simulink model "tractor_mu2018"  (R2018a)
settings: Solver=FixedStepDiscrete  StartTime=0.0  StopTime=30  FixedStep=0.001  RelTol=1e-3
model workspace (MAT data in the model file):
  MCOS : class17 (value not decoded)
undefined symbols (not defined in the file): A, a, B, b, C, D, DiscIntNeverNeededParam, Iz, K, k1, K1, k2, K2, L1, L2, m, magnitude, Phi, Sample_time, Steer_Ratio
libraries: simulink x39, Solver_SF x1, dsparch4 x1
(part 2 of 5)

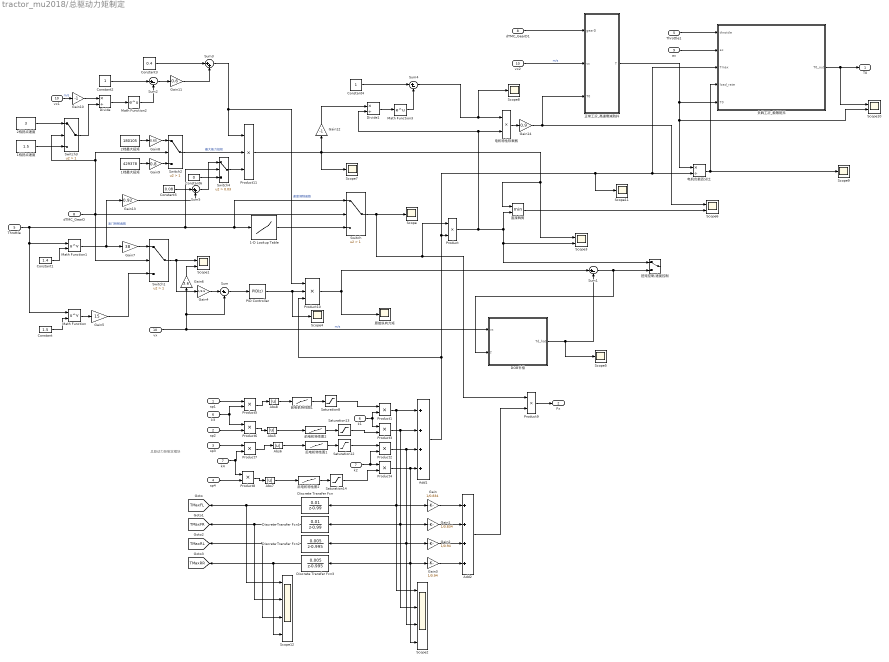
== system tractor_mu2018/总驱动力矩制定 ==
  note: 总驱动力矩制定模块
  sp1 : Inport
  sp2 : Inport  Port=2
  sp3 : Inport  Port=3
  sp4 : Inport  Port=4
  Throttle : Inport  Port=5
  k1 : Inport  Port=6
  k2 : Inport  Port=7
  dTMC_GearD : Inport  Port=8
  ax : Inport  Port=9
  vx : Inport  Port=10
  1-D Lookup Table : Lookup_n-D  NumberOfTableDimensions=1  BreakpointsForDimension1=[0 0.1 0.2 0.3 0.4 0.5 0.6 0.7 0.8 0.9 1]  Table=[0 0.02 0.04 0.09 0.14 0.23 0.32 0.46 0.6 0.8 1]  InternalRulePriority=Speed  RndMeth=Simplest  InputSameDT=on
  1档拐点速度 : Constant  Value=1.5
  1档最大扭矩 : Constant  Value=429378
  2档拐点速度 : Constant  Value=3
  2档最大扭矩 : Constant  Value=180105
  Abs{5..8} (4 alike) : Abs
  Add1 : Sum  Inputs=++++
  Add2 : Sum  Inputs=++++
  Constant : Constant  Value=1.5
  Constant1 : Constant  Value=1.4
  Constant2 : Constant
  Constant3 : Constant  Value=0.4
  Constant4 : Constant
  Constant5 : Constant  Value=0.08
  Constant6 : Constant  Value=0
  DOB补偿 : Subsystem
  Discrete Transfer Fcn : DiscreteTransferFcn  Numerator=[0.01]  Denominator=[1 -0.99]
  Discrete Transfer Fcn1 : DiscreteTransferFcn  Numerator=[0.01]  Denominator=[1 -0.99]
  Discrete Transfer Fcn2 : DiscreteTransferFcn  Numerator=[0.005]  Denominator=[1 -0.995]
  Discrete Transfer Fcn3 : DiscreteTransferFcn  Numerator=[0.005]  Denominator=[1 -0.995]
  Divide : Product  Inputs=*/
  Divide1 : Product  Inputs=*/
  Gain : Gain  Gain=1/0.834
  Gain1 : Gain  Gain=1/0.834
  Gain10 : Gain  Gain=-1
  Gain11 : Gain  Gain=0.6
  Gain12 : Gain  Gain=-1
  Gain13 : Gain  Gain=0.92
  Gain14 : Gain  Gain=0.9
  Gain2 : Gain  Gain=1/0.94
  Gain3 : Gain  Gain=1/0.94
  Gain4 : Gain  Gain=1/3.6
  Gain5 : Gain  Gain=15
  Gain6 : Gain  Gain=3.6
  Gain7 : Gain  Gain=38
  Gain8 : Gain  Gain=0.65
  Gain9 : Gain  Gain=0.8
  Math Function : Math  Operator=pow  SaturateOnIntegerOverflow=on
  Math Function1 : Math  Operator=pow  SaturateOnIntegerOverflow=on
  Math Function2 : Math  SaturateOnIntegerOverflow=on
  Math Function3 : Math  SaturateOnIntegerOverflow=on
  PID Controller : simulink/Continuous/PID Controller  Controller=PID  Form=Parallel  TimeDomain=Discrete-time  SampleTime=-1  IntegratorMethod=Forward Euler  FilterMethod=Forward Euler  ControllerParametersSource=internal  P=0.3  I=0.1  D=0  N=100  UseFilter=on  TunerSelectOption=Transfer Function Based (PID Tuner App)  InitialConditionSource=internal  InitialConditionForIntegrator=0  InitialConditionForFilter=0  DifferentiatorICPrevScaledInput=0  ExternalReset=none  TrackingMode=off  Kt=1  LimitOutput=on  UpperSaturationLimit=1  LowerSaturationLimit=0  LinearizeAsGain=on  AntiWindupMode=none  Kb=1  POutMin=[]  POutMax=[]  IOutMin=[]  IOutMax=[]  DOutMin=[]  DOutMax=[]  NOutMin=[]  NOutMax=[]  SumOutMin=[]  SumOutMax=[]  SaturationOutMin=[]  SaturationOutMax=[]  PParamMin=[]  PParamMax=[]  IParamMin=[]  IParamMax=[]  DParamMin=[]  DParamMax=[]  NParamMin=[]  NParamMax=[]  KbParamMin=[]  KbParamMax=[]  KtParamMin=[]  KtParamMax=[]  KbOutMin=[]  KbOutMax=[]  KtOutMin=[]  KtOutMax=[]  IntegratorOutMin=[]  IntegratorOutMax=[]  FilterOutMin=[]  FilterOutMax=[]  SumI1OutMin=[]  SumI1OutMax=[]  SumI2OutMin=[]  SumI2OutMax=[]  SumI3OutMin=[]  SumI3OutMax=[]  SumDOutMin=[]  SumDOutMax=[]  DifferentiatorOutMin=[]  DifferentiatorOutMax=[]  FilterDiffOutCoefMin=[]  FilterDiffOutCoefMax=[]  ReciprocalOutMin=[]  ReciprocalOutMax=[]  SumDenOutMin=[]  SumDenOutMax=[]  SumNumOutMin=[]  SumNumOutMax=[]  DivideOutMin=[]  DivideOutMax=[]  IntegratorContinuousStateAttributes=''  IntegratorStateMustResolveToSignalObject=off  IntegratorRTWStateStorageClass=Auto  FilterContinuousStateAttributes=''  FilterStateMustResolveToSignalObject=off  FilterRTWStateStorageClass=Auto
  Product{,1..9} (10 alike) : Product
  Product10 : Product  Inputs=3
  Product11 : Product  Inputs=3
  Saturation12 : Saturate  UpperLimit=1800  LowerLimit=0
  Saturation13 : Saturate  UpperLimit=1100  LowerLimit=0
  Saturation14 : Saturate  UpperLimit=1800  LowerLimit=0
  Saturation8 : Saturate  UpperLimit=1100  LowerLimit=0
  Scope{,4..5,7..9,11} (7 alike) : Scope
  Scope{1,3,6,10} (4 alike) : Scope  NumInputPorts=2
  Scope12 : Scope  NumInputPorts=4
  Scope2 : Scope  NumInputPorts=4
  Sum{,1..2,4} (4 alike) : Sum  Inputs=|+-
  Sum3 : Sum  Inputs=|++
  Sum5 : Sum  Inputs=|++
  Switch{,1..3} (4 alike) : Switch  Criteria=u2 > Threshold  Threshold=1
  Switch4 : Switch  Criteria=u2 > Threshold  Threshold=0.03
  Throttle1 : InportShadow  Port=5
  dTMC_GearD1 : InportShadow  Port=8
  k3 : InportShadow  Port=6
  k4 : InportShadow  Port=7
  vx1 : InportShadow  Port=10
  vx2 : InportShadow  Port=10
  前电机特性图1 : Lookup_n-D  NumberOfTableDimensions=1  BreakpointsForDimension1=[0;600;900;1200;1500;1800;2104;2402;2701;3001;3302;3600;3901;4200;4501;4801;5000;5001]  Table=[1116;1107;1102;1099;1101;913;734;611;523;456;403;363;327;305;278;253;240;0]  InternalRulePriority=Speed  OutMin=0  OutMax=1200  RndMeth=Simplest  InputSameDT=on
  前电机特性图2 : Lookup_n-D  NumberOfTableDimensions=1  BreakpointsForDimension1=[0;600;900;1200;1500;1800;2104;2402;2701;3001;3302;3600;3901;4200;4501;4801;5000;5001]  Table=[1116;1107;1102;1099;1101;913;734;611;523;456;403;363;327;305;278;253;240;0]  InternalRulePriority=Speed  OutMin=0  OutMax=1200  RndMeth=Simplest  InputSameDT=on
  原始纵向力矩 : Scope
  后电机特性图1 : Lookup_n-D  NumberOfTableDimensions=1  BreakpointsForDimension1=[0;299;599.6;899.7;1200;1500;1800;2099;2399.4;2698.5;2998.1;3300;3599;3899;4197.8;4201]  Table=[1868;1868.3;1868.6;1844.3;1842.3;1763.9;1516.4;1277.9;1098.6;954;839.4;727;645.7;585.53;529.7;0]  InternalRulePriority=Speed  OutMin=[0]  OutMax=[1800]  RndMeth=Simplest  InputSameDT=on
  后电机特性图2 : Lookup_n-D  NumberOfTableDimensions=1  BreakpointsForDimension1=[0;500;1000;1200;1600;2000;2800;3200;3600;4200;4201]  Table=[1800;1800;1800;1800;1700;1360;900;750;650;520;0]  InternalRulePriority=Speed  OutMin=[0]  OutMax=[1800]  RndMeth=Simplest  InputSameDT=on
  扭矩控制/速度控制 : ManualSwitch
  正常工况_高速衰减防抖 : Subsystem
  电机特性软裁剪 : Product
  电机负载百分比 : Product  Inputs=*/
  直接裁剪 : MinMax  Inputs=2
  负载工况_极限防抖 : Stateflow chart  TreatAsAtomicUnit=on
  T0 : Outport
  Fx : Outport  Port=2
  tag scope: TMaxFL=global, TMaxFR=global, TMaxRL=global, TMaxRR=global
  wires:
  sp3/1 -> Product7/1
  Saturation8/1 -> Product1/1
  前电机特性图2/1 -> Saturation13/1
  后电机特性图1/1 -> Saturation12/1
  sp1/1 -> Product5/1
  sp4/1 -> Product8/2
  Abs7/1 -> 后电机特性图2/1
  Product2/1 -> Discrete Transfer Fcn2/1, Scope2/3, Gain2/1, Add1/3
  前电机特性图1/1 -> Saturation8/1
  sp2/1 -> Product6/2
  Product3/1 -> Add1/2, Discrete Transfer Fcn1/1, Scope2/2, Gain1/1
  后电机特性图2/1 -> Saturation14/1
  Saturation12/1 -> Product2/1
  Abs5/1 -> 前电机特性图2/1
  Abs6/1 -> 后电机特性图1/1
  Abs8/1 -> 前电机特性图1/1
  k1/1 -> Product3/1, Product1/2
  Saturation13/1 -> Product3/2
  k2/1 -> Product4/1, Product2/2
  Saturation14/1 -> Product4/2
  Product4/1 -> Discrete Transfer Fcn3/1, Scope2/4, Gain3/1, Add1/4
  Product/1 -> Divide1/2, 电机特性软裁剪/2, 直接裁剪/2, Scope3/2, 扭矩控制/速度控制/1
  k3/1 -> Product6/1, Product5/2
  Product5/1 -> Abs8/1
  Product6/1 -> Abs5/1
  k4/1 -> Product8/1, Product7/2
  Product7/1 -> Abs6/1
  Product8/1 -> Abs7/1
  1-D Lookup Table/1 -> Switch/3
  Gain/1 -> Add2/1
  Gain1/1 -> Add2/2
  Gain2/1 -> Add2/3
  Gain3/1 -> Add2/4
  Add2/1 -> Product9/2
  Product9/1 -> Fx/1
  Throttle/1 -> Math Function/1, Math Function1/1, Switch4/2, Switch/1, 1-D Lookup Table/1
  Constant/1 -> Math Function/2
  Math Function/1 -> Gain5/1
  Gain5/1 -> Switch1/3
  Constant1/1 -> Math Function1/2
  Gain7/1 -> Switch1/1
  Math Function1/1 -> Gain13/1, Gain7/1  "油门映射函数"
  Switch1/1 -> Gain4/1, Scope1/1
  Gain4/1 -> Sum/1
  vx/1 -> Sum/2, Gain6/1, DOB补偿/1(vx)  "m/s"
  Switch/1 -> Product9/1, Product/1, Scope/1
  Sum/1 -> PID Controller/1
  PID Controller/1 -> Scope4/1, Product10/2
  Product10/1 -> Sum1/1, 原始纵向力矩/1
  Gain6/1 -> Scope1/2
  Sum1/1 -> DOB补偿/2(T), 扭矩控制/速度控制/2
  DOB补偿/1(Td_hat) -> Scope5/1, Sum1/2
  1档最大扭矩/1 -> Gain9/1
  2档最大扭矩/1 -> Gain8/1
  Gain8/1 -> Switch2/1
  Gain9/1 -> Switch2/3
  Switch2/1 -> Product11/2  "最大能力扭矩"
  Constant2/1 -> Sum2/1
  Math Function2/1 -> Sum2/2
  1档拐点速度/1 -> Switch3/3
  2档拐点速度/1 -> Switch3/1
  dTMC_GearD/1 -> Switch3/2, Switch2/2, Switch1/2, Switch/2
  vx1/1 -> Gain10/1  "m/s"
  Switch3/1 -> Divide/2
  Gain10/1 -> Divide/1
  Divide/1 -> Math Function2/1
  Sum2/1 -> Gain11/1
  Constant3/1 -> Sum3/1
  Gain11/1 -> Sum3/2
  Sum3/1 -> Product10/1, Product11/1  "速度调制函数"
  Constant4/1 -> Sum4/1
  Math Function3/1 -> Sum4/2
  Divide1/1 -> Math Function3/1
  Gain12/1 -> Divide1/1
  Sum4/1 -> Scope8/1, 电机特性软裁剪/1
  Product11/1 -> Scope7/1, 直接裁剪/1, Scope3/1, Gain12/1
  Sum5/1 -> Switch4/1
  Gain13/1 -> Sum5/2
  Constant5/1 -> Sum5/1
  Switch4/1 -> Product11/3
  Constant6/1 -> Switch4/3
  电机特性软裁剪/1 -> Gain14/1
  直接裁剪/1 -> Scope6/2
  Product1/1 -> Discrete Transfer Fcn/1, Scope2/1, Gain/1, Add1/1
  dTMC_GearD1/1 -> 正常工况_高速衰减防抖/1(gearD)
  vx2/1 -> 正常工况_高速衰减防抖/2(vx)  "m/s"
  Throttle1/1 -> 负载工况_极限防抖/1(throttle)
  ax/1 -> 负载工况_极限防抖/2(ax)
  Add1/1 -> Scope11/1, 负载工况_极限防抖/3(Tmax), 电机负载百分比/2, Product/2, Product10/3
  正常工况_高速衰减防抖/1(T) -> 负载工况_极限防抖/5(T0), Scope10/2, 电机负载百分比/1
  电机负载百分比/1 -> 负载工况_极限防抖/4(load_rate), Scope9/1
  负载工况_极限防抖/1(T0_out) -> Scope10/1, T0/1
  Discrete Transfer Fcn/1 -> Scope12/1, [TMaxFL]
  Discrete Transfer Fcn1/1 -> Scope12/2, [TMaxFR]
  Discrete Transfer Fcn2/1 -> Scope12/3, [TMaxRL]
  Discrete Transfer Fcn3/1 -> Scope12/4, [TMaxRR]
  Gain14/1 -> Scope6/1, 正常工况_高速衰减防抖/3(T0)

== system tractor_mu2018/挡位与刹车处理1 ==
  dTMC_GearD : Inport
  Constant6 : Constant  Value=15.88
  Constant7 : Constant  Value=30.6204
  Constant8 : Constant  Value=63.52
  Constant9 : Constant  Value=80.454
  Switch2 : Switch  Criteria=u2 > Threshold  Threshold=1
  Switch3 : Switch  Criteria=u2 > Threshold  Threshold=1
  spdratio_F : Outport
  spdratio_R : Outport  Port=2
  wires:
  Switch3/1 -> spdratio_R/1
  Constant9/1 -> Switch3/3
  Switch2/1 -> spdratio_F/1
  Constant8/1 -> Switch2/3
  dTMC_GearD/1 -> Switch3/2, Switch2/2
  Constant6/1 -> Switch2/1
  Constant7/1 -> Switch3/1

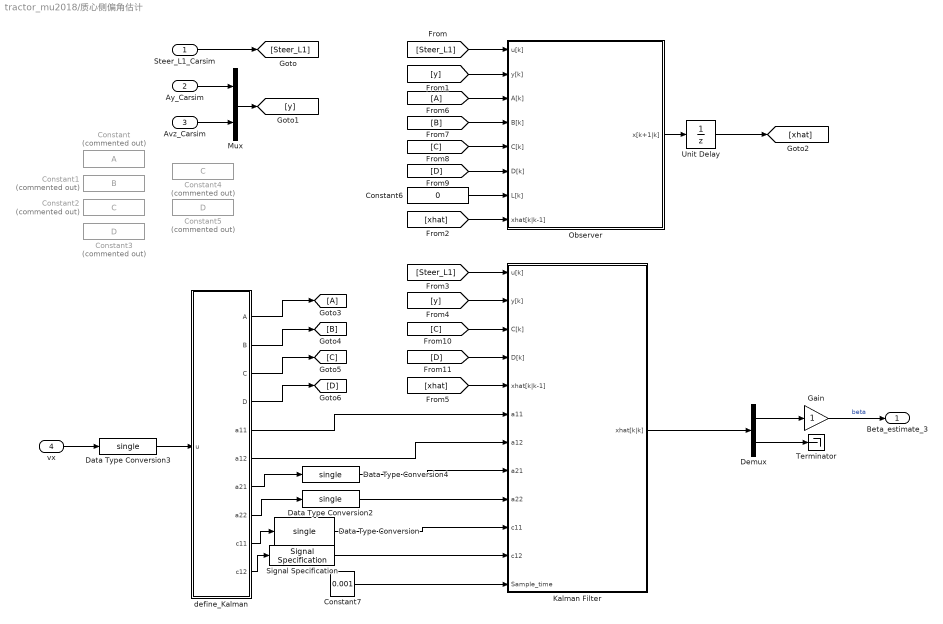
== system tractor_mu2018/质心侧偏角估计 ==
  Steer_L1_Carsim : Inport
  Ay_Carsim : Inport  Port=2
  Avz_Carsim : Inport  Port=3
  vx : Inport  Port=4
  Constant : Constant  Commented=on  Value=A
  Constant1 : Constant  Commented=on  Value=B
  Constant2 : Constant  Commented=on  Value=C
  Constant3 : Constant  Commented=on  Value=D
  Constant4 : Constant  Commented=on  Value=C
  Constant5 : Constant  Commented=on  Value=D
  Constant6 : Constant  Value=0
  Constant7 : Constant  Value=0.001  OutDataTypeStr=single
  Data Type Conversion{,2..4} (4 alike) : DataTypeConversion  OutDataTypeStr=single
  Demux : Demux  Outputs=2
  Gain : Gain
  Kalman Filter : Subsystem
  Mux : Mux  Inputs=2
  Observer : Subsystem
  Signal Specification : SignalSpecification  OutDataTypeStr=single
  Terminator : Terminator
  Unit Delay : UnitDelay  SampleTime=-1  HasFrameUpgradeWarning=on
  define_Kalman : MATLAB Function  TreatAsAtomicUnit=on
  Beta_estimate_3 : Outport
  wires:
  Steer_L1_Carsim/1 -> [Steer_L1]
  Ay_Carsim/1 -> Mux/1
  Avz_Carsim/1 -> Mux/2
  Mux/1 -> [y]
  [Steer_L1] -> Observer/1(u[k])
  [y] -> Observer/2(y[k])
  Observer/1(x[k+1|k]) -> Unit Delay/1
  Unit Delay/1 -> [xhat]
  [xhat] -> Observer/8(xhat[k|k-1])
  [Steer_L1] -> Kalman Filter/1(u[k])
  [y] -> Kalman Filter/2(y[k])
  [xhat] -> Kalman Filter/5(xhat[k|k-1])
  Demux/1 -> Gain/1
  Demux/2 -> Terminator/1
  Constant6/1 -> Observer/7(L[k])
  vx/1 -> Data Type Conversion3/1
  define_Kalman/1(A) -> [A]
  define_Kalman/2(B) -> [B]
  define_Kalman/3(C) -> [C]
  define_Kalman/4(D) -> [D]
  [A] -> Observer/3(A[k])
  [B] -> Observer/4(B[k])
  [C] -> Observer/5(C[k])
  [D] -> Observer/6(D[k])
  [C] -> Kalman Filter/3(C[k])
  [D] -> Kalman Filter/4(D[k])
  Constant7/1 -> Kalman Filter/12(Sample_time)
  define_Kalman/10(c12) -> Signal Specification/1
  define_Kalman/9(c11) -> Data Type Conversion/1
  define_Kalman/8(a22) -> Data Type Conversion2/1
  define_Kalman/6(a12) -> Kalman Filter/7(a12)
  define_Kalman/5(a11) -> Kalman Filter/6(a11)
  Signal Specification/1 -> Kalman Filter/11(c12)
  Data Type Conversion3/1 -> define_Kalman/1(u)
  define_Kalman/7(a21) -> Data Type Conversion4/1
  Data Type Conversion2/1 -> Kalman Filter/9(a22)
  Data Type Conversion/1 -> Kalman Filter/10(c11)
  Kalman Filter/1(xhat[k|k]) -> Demux/1
  Data Type Conversion4/1 -> Kalman Filter/8(a21)
  Gain/1 -> Beta_estimate_3/1  "beta"

== system tractor_mu2018/质心侧偏角滑模观测器估计 ==
  Steer_L1_Carsim : Inport
  Avz_Carsim : Inport  Port=2
  vx : Inport  Port=3
  Subsystem : Subsystem
  Subsystem1 : Subsystem  Commented=on
  delta_f : Gain  Gain=1/Steer_Ratio
  beta_est : Outport
  gamma_est : Outport  Port=2
  vy_hat_out : Outport  Port=3
  wires:
  Steer_L1_Carsim/1 -> delta_f/1
  Avz_Carsim/1 -> Subsystem/1(Avz_Carsim)
  vx/1 -> Subsystem/2(vx)
  delta_f/1 -> Subsystem/3(delta_f)
  Subsystem/1(beta_est) -> beta_est/1
  Subsystem/2(gamma_est) -> gamma_est/1
  Subsystem/3(vy_hat_output) -> vy_hat_out/1

== system tractor_mu2018/质心侧偏角观测 ==
  前轮转角 : Inport
  前轮纵向力 : Inport  Port=2
  后轮纵向力 : Inport  Port=3
  纵向速度 : Inport  Port=4
  横摆角速度 : Inport  Port=5
  Demux : Demux  Outputs=3
  Gain : Gain  Gain=0.001
  MATLAB Function : MATLAB Function  TreatAsAtomicUnit=on
  Mux : Mux  Inputs=3
  Mux1 : Mux  Inputs=2
  Scope : Scope
  Scope1 : Scope
  Sum : Sum  Inputs=|++
  Sum1 : Sum  Inputs=|+-
  Unit Delay : UnitDelay  InitialCondition=[0.1;0;0]  SampleTime=0.001  HasFrameUpgradeWarning=on
  Unit Delay1 : UnitDelay  InitialCondition=[0.1;0;0]  SampleTime=0.001  HasFrameUpgradeWarning=on
  估计横摆角速度 : Scope
  估计纵向速度 : Scope
  侧偏角估计 : Scope
  侧偏角 : Outport
  纵向速度估计 : Outport  Port=2
  横摆角速度估计 : Outport  Port=3
  wires:
  MATLAB Function/1(x_dot) -> Scope1/1, Gain/1
  Gain/1 -> Sum/1
  Unit Delay/1 -> Sum/2
  Sum/1 -> Unit Delay1/1, Demux/1, Unit Delay/1
  Demux/2 -> 侧偏角估计/1, 侧偏角/1
  Demux/1 -> 纵向速度估计/1, 估计纵向速度/1
  Demux/3 -> 横摆角速度估计/1, 估计横摆角速度/1
  前轮转角/1 -> Mux/1
  前轮纵向力/1 -> Mux/2
  后轮纵向力/1 -> Mux/3
  Mux/1 -> MATLAB Function/2(u)
  纵向速度/1 -> Mux1/1
  横摆角速度/1 -> Mux1/2
  Mux1/1 -> Sum1/1, MATLAB Function/3(z_meas)
  MATLAB Function/2(z_hat) -> Sum1/2
  Sum1/1 -> Scope/1
  Unit Delay1/1 -> MATLAB Function/1(x_hat)

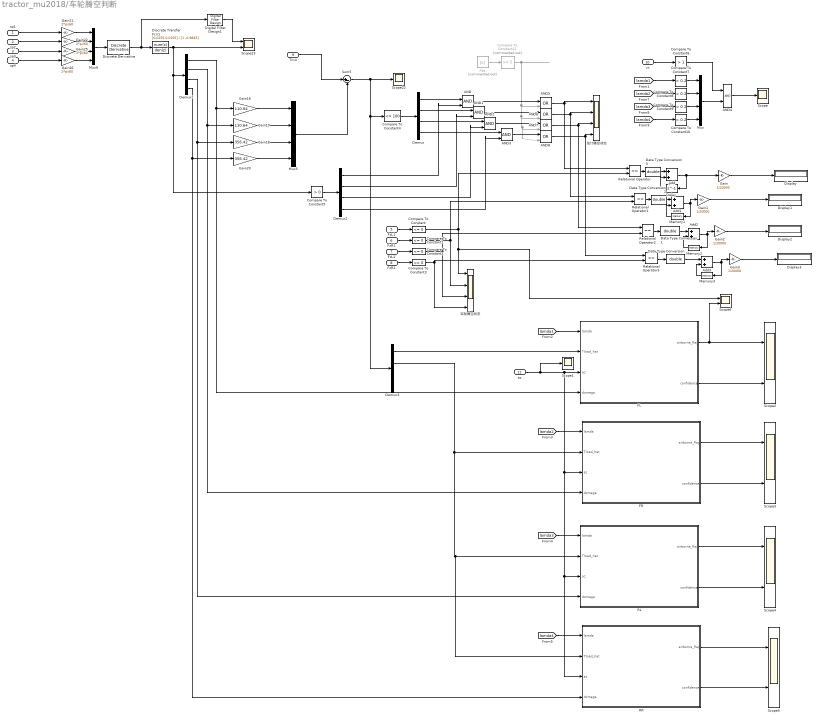
== system tractor_mu2018/车轮腾空判断 ==
  sp1 : Inport
  sp2 : Inport  Port=2
  sp3 : Inport  Port=3
  sp4 : Inport  Port=4
  FzL1 : Inport  Port=5
  FzR1 : Inport  Port=6
  FzL2 : Inport  Port=7
  FzR2 : Inport  Port=8
  Tm4 : Inport  Port=9
  vx : Inport  Port=10
  az : Inport  Port=11
  AND{,1..4} (5 alike) : Logic  IconShape=distinctive  AllPortsSameDT=off  OutDataTypeStr=boolean
  AND{5..8} (4 alike) : Logic  Operator=OR  IconShape=distinctive  AllPortsSameDT=off  OutDataTypeStr=boolean
  Abs : Abs  Commented=on
  Add : Sum
  Add1 : Sum
  Add2 : Sum
  Add3 : Sum  AccumDataTypeStr=double
  Compare To Constant{,1..3} (4 alike) : simulink/Logic and Bit Operations/Compare To Constant  relop=<=  const=0  OutDataTypeStr=boolean
  Compare To Constant{7..10} (4 alike) : simulink/Logic and Bit Operations/Compare To Constant  relop=>  const=0.2  OutDataTypeStr=boolean
  Compare To Constant11 : simulink/Logic and Bit Operations/Compare To Constant  Commented=on  relop=>=  const=5  OutDataTypeStr=boolean
  Compare To Constant4 : simulink/Logic and Bit Operations/Compare To Constant  relop=<=  const=100  OutDataTypeStr=boolean
  Compare To Constant5 : simulink/Logic and Bit Operations/Compare To Constant  relop=>  const=0  OutDataTypeStr=boolean
  Compare To Constant6 : simulink/Logic and Bit Operations/Compare To Constant  relop=>  const=1  OutDataTypeStr=boolean
  Data Type Conversion{,1..3} (4 alike) : DataTypeConversion  OutDataTypeStr=double
  Delay : Delay  DelayLength=1
  Demux{,1..3} (4 alike) : Demux
  Digital Filter Design1 : dsparch4/Digital Filter Design  mwdsp_browser_bugfix_var=off
  Discrete Transfer Fcn1 : DiscreteTransferFcn  Numerator=[0.0155 0.0155]  Denominator=[1 -0.9845]
  Discrete Derivative : simulink/Discrete/Discrete Derivative  gainval=1.0  ICPrevScaledInput=0.0  OutMin=[]  OutMax=[]  OutDataType=fixdt(1, 16)  OutScaling=2^-10  DoSatur=off
  Display{,1..3} (4 alike) : Display
  FL : Stateflow chart  TreatAsAtomicUnit=on
  FR : Stateflow chart  TreatAsAtomicUnit=on
  Gain{,1..3} (4 alike) : Gain  Gain=1/20000
  Gain16 : Gain  Gain=110.64
  Gain18 : Gain  Gain=356.42
  Gain19 : Gain  Gain=110.64
  Gain20 : Gain  Gain=356.42
  Gain{21..22,25..26} (4 alike) : Gain  Gain=2*pi/60
  Memory1 : Memory
  Memory2 : Memory
  Memory3 : Memory
  Mux : Mux
  Mux5 : Mux
  Mux6 : Mux
  RL : Stateflow chart  TreatAsAtomicUnit=on
  RR : Stateflow chart  TreatAsAtomicUnit=on
  Relational Operator{,1..3} (4 alike) : RelationalOperator  Operator===  OutDataTypeStr=boolean  RndMeth=Simplest
  Scope : Scope
  Scope1 : Scope
  Scope{2..6,23} (6 alike) : Scope  NumInputPorts=2
  Scope22 : Scope
  Sum5 : Sum  Inputs=|+-
  估计腾空状态 : Scope  NumInputPorts=4
  实际腾空状态 : Scope  NumInputPorts=4
  wires:
  Digital Filter Design1/1 -> Scope23/1
  Compare To Constant2/1 -> Relational Operator2/2, 实际腾空状态/3
  sp2/1 -> Gain22/1
  Discrete Transfer Fcn1/1 -> Compare To Constant5/1, Demux1/1, Scope23/2
  Compare To Constant3/1 -> Relational Operator3/2, 实际腾空状态/4
  Compare To Constant/1 -> Relational Operator/2, Scope6/1, 实际腾空状态/1
  FzL1/1 -> Compare To Constant/1
  Gain21/1 -> Mux6/1
  Mux5/1 -> Sum5/2
  Tm4/1 -> Sum5/1
  Mux6/1 -> Discrete Derivative/1
  Gain19/1 -> Mux5/2
  Gain26/1 -> Mux6/4
  Discrete Derivative/1 -> Digital Filter Design1/1, Discrete Transfer Fcn1/1
  Gain22/1 -> Mux6/2
  Compare To Constant1/1 -> Relational Operator1/2, 实际腾空状态/2
  Gain18/1 -> Mux5/3
  Gain25/1 -> Mux6/3
  Gain20/1 -> Mux5/4
  FzR2/1 -> Compare To Constant3/1
  Demux1/1 -> FL/4(domega), Gain16/1
  FzL2/1 -> Compare To Constant2/1
  Gain16/1 -> Mux5/1
  FzR1/1 -> Compare To Constant1/1
  sp4/1 -> Gain26/1
  sp1/1 -> Gain21/1
  sp3/1 -> Gain25/1
  Compare To Constant4/1 -> Demux/1
  Compare To Constant5/1 -> Demux2/1
  Demux/1 -> AND/1
  Demux2/1 -> AND/2
  Demux/2 -> AND1/1
  Demux2/2 -> AND1/2
  Demux/3 -> AND2/1
  Demux2/3 -> AND2/2
  Demux/4 -> AND3/1
  Demux2/4 -> AND3/2
  AND8/1 -> 估计腾空状态/4, Relational Operator3/1
  AND7/1 -> 估计腾空状态/3, Relational Operator2/1
  AND6/1 -> 估计腾空状态/2, Relational Operator1/1
  AND5/1 -> 估计腾空状态/1, Relational Operator/1
  Relational Operator/1 -> Data Type Conversion3/1
  Gain/1 -> Display/1
  Gain1/1 -> Display1/1
  Gain2/1 -> Display2/1
  Gain3/1 -> Display3/1
  Add/1 -> Delay/1, Gain/1
  Delay/1 -> Add/2
  Relational Operator1/1 -> Data Type Conversion2/1
  Add1/1 -> Memory1/1, Gain1/1
  Memory1/1 -> Add1/2
  Relational Operator2/1 -> Data Type Conversion1/1
  Memory2/1 -> Add2/2
  Add2/1 -> Gain2/1, Memory2/1
  Relational Operator3/1 -> Data Type Conversion/1
  Memory3/1 -> Add3/2
  Add3/1 -> Memory3/1, Gain3/1
  Data Type Conversion/1 -> Add3/1
  Data Type Conversion1/1 -> Add2/1
  Data Type Conversion2/1 -> Add1/1
  Data Type Conversion3/1 -> Add/1
  vx/1 -> Compare To Constant6/1
  Compare To Constant6/1 -> AND4/1
  [lamda4] -> Compare To Constant10/1
  [lamda3] -> Compare To Constant9/1
  [lamda2] -> Compare To Constant8/1
  [lamda1] -> Compare To Constant7/1
  Compare To Constant7/1 -> Mux/1
  Compare To Constant8/1 -> Mux/2
  Compare To Constant9/1 -> Mux/3
  Compare To Constant10/1 -> Mux/4
  Mux/1 -> AND4/2
  AND4/1 -> Scope/1
  ? -> Abs/1
  Abs/1 -> Compare To Constant11/1
  Compare To Constant11/1 -> AND8/2, AND7/2, AND6/2, AND5/2
  AND/1 -> AND5/1
  AND1/1 -> AND6/1
  AND2/1 -> AND7/1
  AND3/1 -> AND8/1
  [lamda1] -> FL/1(lamda)
  Demux3/1 -> FL/2(Tload_hat)
  Sum5/1 -> Demux3/1, Compare To Constant4/1, Scope22/1
  az/1 -> Scope1/1, RR/3(az), RL/3(az), FR/3(az), FL/3(az)
  FL/1(airborne_flag) -> Scope6/2, Scope2/1
  FL/2(confidence) -> Scope2/2
  [lamda2] -> FR/1(lamda)
  [lamda3] -> RL/1(lamda)
  [lamda4] -> RR/1(lamda)
  Demux3/2 -> RR/2(Tload_hat), RL/2(Tload_hat), FR/2(Tload_hat)
  Demux1/2 -> FR/4(domega), Gain19/1
  Demux1/3 -> RL/4(domega), Gain18/1
  Demux1/4 -> RR/4(domega), Gain20/1
  FR/1(airborne_flag) -> Scope3/1
  FR/2(confidence) -> Scope3/2
  RL/1(airborne_flag) -> Scope4/1
  RL/2(confidence) -> Scope4/2
  RR/1(airborne_flag) -> Scope5/1
  RR/2(confidence) -> Scope5/2

== system tractor_mu2018/软土分配策略 ==
  sp_all : Inport
  vx(m/s) : Inport  Port=2
  st : Inport  Port=3
  Tmax : Inport  Port=4
  base_Torque : Inport  Port=5
  Constant : Constant  OutDataTypeStr=single
  Data Type Conversion : DataTypeConversion  OutDataTypeStr=single
  Data Type Conversion1 : DataTypeConversion  OutDataTypeStr=single
  Demux : Demux
  Gain : Gain  Gain=0.8  OutDataTypeStr=single
  MATLAB Function : MATLAB Function  TreatAsAtomicUnit=on
  MATLAB Function1 : MATLAB Function  TreatAsAtomicUnit=on
  Mux : Mux
  Mux1 : Mux
  Unit Delay : UnitDelay  SampleTime=-1  HasFrameUpgradeWarning=on
  Tfl_soft : Outport
  Tfr_soft : Outport  Port=2
  Trl_soft : Outport  Port=3
  Trr_soft : Outport  Port=4
  wires:
  vx(m/s)/1 -> MATLAB Function/3(longitudinal_speed_mps)
  st/1 -> MATLAB Function/2(front_steer_angles_deg)
  sp_all/1 -> Data Type Conversion/1
  Data Type Conversion/1 -> MATLAB Function/1(wheel_speeds_rpm)
  Constant/1 -> MATLAB Function/5(drive_torque_enabled)
  base_Torque/1 -> MATLAB Function1/2(baseline_torques_n_m), MATLAB Function/6(baseline_torques_n_m)
  Tmax/1 -> MATLAB Function1/3(wheel_torque_limits_n_m), Gain/1
  Gain/1 -> MATLAB Function/7(wheel_torque_limits_n_m)
  MATLAB Function/1(selected_torques_n_m) -> Data Type Conversion1/1
  Unit Delay/1 -> MATLAB Function/4(applied_torques_n_m)
  Data Type Conversion1/1 -> Unit Delay/1  "Tfl_soft"
  Demux/1 -> Tfl_soft/1
  Demux/2 -> Tfr_soft/1
  Demux/3 -> Trl_soft/1
  Demux/4 -> Trr_soft/1
  [lamda1] -> Mux/1
  [lamda2] -> Mux/2
  [lamda4] -> Mux/4
  [lamda3] -> Mux/3
  Mux/1 -> MATLAB Function1/1(measured_kappa)
  MATLAB Function1/1(torque_l1_n_m) -> Mux1/1
  MATLAB Function1/2(torque_r1_n_m) -> Mux1/2
  MATLAB Function1/3(torque_l2_n_m) -> Mux1/3
  MATLAB Function1/4(torque_r2_n_m) -> Mux1/4
  Mux1/1 -> Demux/1

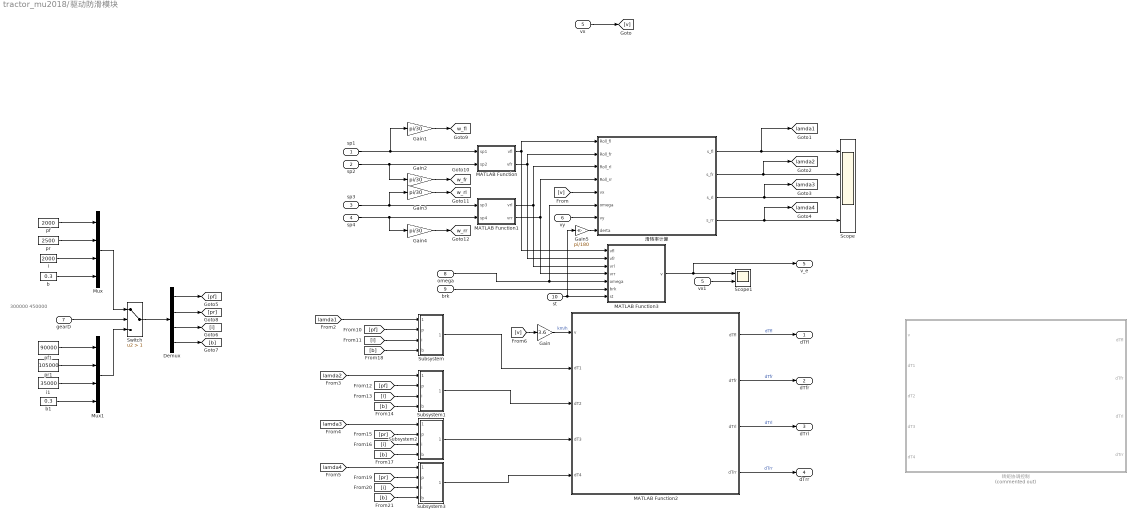
== system tractor_mu2018/驱动防滑模块 ==
  note: 300000
      | 450000
  sp1 : Inport
  sp2 : Inport  Port=2
  sp3 : Inport  Port=3
  sp4 : Inport  Port=4
  vx : Inport  Port=5
  vy : Inport  Port=6
  gearD : Inport  Port=7
  omega : Inport  Port=8
  brk : Inport  Port=9
  st : Inport  Port=10
  Demux : Demux
  Gain : Gain  Gain=3.6
  Gain{1..4} (4 alike) : Gain  Gain=pi/30
  Gain5 : Gain  Gain=pi/180
  MATLAB Function : MATLAB Function  TreatAsAtomicUnit=on
  MATLAB Function1 : MATLAB Function  TreatAsAtomicUnit=on
  MATLAB Function2 : MATLAB Function  TreatAsAtomicUnit=on
  MATLAB Function3 : MATLAB Function  TreatAsAtomicUnit=on
  Mux : Mux
  Mux1 : Mux
  Scope : Scope  NumInputPorts=4
  Scope1 : Scope  NumInputPorts=2
  Subsystem : Subsystem
  Subsystem1 : Subsystem
  Subsystem2 : Subsystem
  Subsystem3 : Subsystem
  Switch : Switch  Criteria=u2 > Threshold  Threshold=1
  b : Constant  Value=0.3
  b1 : Constant  Value=0.3
  i : Constant  Value=2000
  i1 : Constant  Value=35000
  pf : Constant  Value=2000
  pf1 : Constant  Value=90000
  pr : Constant  Value=2500
  pr1 : Constant  Value=105000
  vx1 : InportShadow  Port=5
  滑转率计算 : Subsystem
  转矩协调控制 : Stateflow chart  Commented=on  TreatAsAtomicUnit=on
  dTfl : Outport
  dTfr : Outport  Port=2
  dTrl : Outport  Port=3
  dTrr : Outport  Port=4
  v_e : Outport  Port=5
  tag scope: lamda1=global, lamda2=global, lamda3=global, lamda4=global, w_fl=global, w_fr=global, w_rl=global, w_rr=global
  wires:
  MATLAB Function/2(vfr) -> 滑转率计算/2(Roll_fr), MATLAB Function3/2(vfr)
  MATLAB Function/1(vfl) -> MATLAB Function3/1(vfl), 滑转率计算/1(Roll_fl)
  MATLAB Function1/1(vrl) -> MATLAB Function3/3(vrl), 滑转率计算/3(Roll_rl)
  MATLAB Function1/2(vrr) -> MATLAB Function3/4(vrr), 滑转率计算/4(Roll_rr)
  [v] -> Gain/1
  Gain/1 -> MATLAB Function2/1(v)  "km/h"
  sp1/1 -> Gain1/1, MATLAB Function/1(sp1)
  sp2/1 -> Gain2/1, MATLAB Function/2(sp2)
  sp3/1 -> Gain3/1, MATLAB Function1/1(sp3)
  sp4/1 -> Gain4/1, MATLAB Function1/2(sp4)
  MATLAB Function2/1(dTfl) -> dTfl/1  "dTfl"
  MATLAB Function2/2(dTfr) -> dTfr/1  "dTfr"
  MATLAB Function2/3(dTrl) -> dTrl/1  "dTrl"
  MATLAB Function2/4(dTrr) -> dTrr/1  "dTrr"
  vx/1 -> [v]
  [lamda1] -> Subsystem/1(lamda1)
  Subsystem/1(dT1) -> MATLAB Function2/2(dT1)
  [pf] -> Subsystem/2(p)
  [i] -> Subsystem/3(i)
  [b] -> Subsystem/4(b)
  [b] -> Subsystem1/4(b)
  [i] -> Subsystem1/3(i)
  [pf] -> Subsystem1/2(p)
  Subsystem1/1(dT1) -> MATLAB Function2/3(dT2)
  [lamda2] -> Subsystem1/1(lamda2)
  [lamda3] -> Subsystem2/1(lamda3)
  [pr] -> Subsystem2/2(p)
  [i] -> Subsystem2/3(i)
  [b] -> Subsystem2/4(b)
  Subsystem2/1(dT1) -> MATLAB Function2/4(dT3)
  Subsystem3/1(dT1) -> MATLAB Function2/5(dT4)
  [b] -> Subsystem3/4(b)
  [i] -> Subsystem3/3(i)
  [pr] -> Subsystem3/2(p)
  [lamda4] -> Subsystem3/1(lamda4)
  gearD/1 -> Switch/2
  b/1 -> Mux/4
  i/1 -> Mux/3
  pf/1 -> Mux/1
  pr/1 -> Mux/2
  pr1/1 -> Mux1/2
  pf1/1 -> Mux1/1
  b1/1 -> Mux1/4
  i1/1 -> Mux1/3
  Mux/1 -> Switch/1
  Mux1/1 -> Switch/3
  Switch/1 -> Demux/1
  Demux/1 -> [pf]
  Demux/2 -> [pr]
  Demux/3 -> [i]
  Demux/4 -> [b]
  omega/1 -> 滑转率计算/6(omega), MATLAB Function3/5(omega)
  brk/1 -> MATLAB Function3/6(brk)
  st/1 -> Gain5/1, MATLAB Function3/7(st)
  MATLAB Function3/1(v) -> v_e/1, Scope1/1
  vx1/1 -> Scope1/2
  Gain1/1 -> [w_fl]
  Gain2/1 -> [w_fr]
  Gain3/1 -> [w_rl]
  Gain4/1 -> [w_rr]
  Gain5/1 -> 滑转率计算/8(derta)
  vy/1 -> 滑转率计算/7(vy)
  [v] -> 滑转率计算/5(vx)
  滑转率计算/1(s_fl) -> [lamda1], Scope/1
  滑转率计算/2(s_fr) -> [lamda2], Scope/2
  滑转率计算/3(s_rl) -> [lamda3], Scope/3
  滑转率计算/4(s_rr) -> [lamda4], Scope/4

== system tractor_mu2018/Dugoff轮胎模型/alpha_lamda ==
  vx : Inport
  vy : Inport  Port=2
  wz : Inport  Port=3
  delta_fl : Inport  Port=4
  delta_fr : Inport  Port=5
  w_fl : Inport  Port=6
  w_fr : Inport  Port=7
  w_rl : Inport  Port=8
  w_rr : Inport  Port=9
  Scope : Scope  NumInputPorts=4
  alpha : Subsystem
  lamda : Subsystem
  lamda_fl : Outport
  lamda_fr : Outport  Port=2
  lamda_rl : Outport  Port=3
  lamda_rr : Outport  Port=4
  alpha_fl : Outport  Port=5
  alpha_fr : Outport  Port=6
  alpha_rl : Outport  Port=7
  alpha_rr : Outport  Port=8
  wires:
  lamda/3(lamda_rl) -> Scope/3, lamda_rl/1
  lamda/4(lamda_rr) -> Scope/4, lamda_rr/1
  lamda/2(lamda_fr) -> Scope/2, lamda_fr/1
  lamda/1(lamda_fl) -> Scope/1, lamda_fl/1
  w_rr/1 -> lamda/9(w_rr)
  w_rl/1 -> lamda/8(w_rl)
  w_fr/1 -> lamda/7(w_fr)
  w_fl/1 -> lamda/6(w_fl)
  delta_fr/1 -> alpha/5(delta_fr), lamda/5(delta_fr)
  delta_fl/1 -> alpha/4(delta_fl), lamda/4(delta_fl)
  wz/1 -> alpha/3(wz), lamda/3(wz)
  vy/1 -> alpha/2(vy), lamda/2(vy)
  vx/1 -> alpha/1(vx), lamda/1(vx)
  alpha/4(alpha_rr) -> alpha_rr/1
  alpha/3(alpha_rl) -> alpha_rl/1
  alpha/2(alpha_fr) -> alpha_fr/1
  alpha/1(alpha_fl) -> alpha_fl/1

== system tractor_mu2018/Dugoff轮胎模型/pac2002 ==
  lamda_fl : Inport
  lamda_fr : Inport  Port=2
  lamda_rl : Inport  Port=3
  lamda_rr : Inport  Port=4
  alpha_fl : Inport  Port=5
  alpha_fr : Inport  Port=6
  alpha_rl : Inport  Port=7
  alpha_rr : Inport  Port=8
  Fz_fl : Inport  Port=9
  Fz_rl : Inport  Port=10
  Fz_fr : Inport  Port=11
  Fz_rr : Inport  Port=12
  mu : Inport  Port=13
  Demux : Demux
  Gain{8..11} (4 alike) : Gain  Gain=-1
  fl_dugoff : MATLAB Function  TreatAsAtomicUnit=on
  fr_dugoff : MATLAB Function  TreatAsAtomicUnit=on
  rl_dugoff : MATLAB Function  TreatAsAtomicUnit=on
  rr_dugoff : MATLAB Function  TreatAsAtomicUnit=on
  Fx_fl : Outport
  Fx_fr : Outport  Port=2
  Fx_rl : Outport  Port=3
  Fx_rr : Outport  Port=4
  Fy_fl : Outport  Port=5
  Fy_fr : Outport  Port=6
  Fy_rl : Outport  Port=7
  Fy_rr : Outport  Port=8
  wires:
  alpha_fl/1 -> fl_dugoff/4(alpha)
  Fz_fl/1 -> fl_dugoff/1(Fz)
  alpha_rr/1 -> rr_dugoff/4(alpha)
  Fz_rr/1 -> rr_dugoff/1(Fz)
  [u_fl] -> fl_dugoff/2(u)
  [u_fr] -> fr_dugoff/2(u)
  alpha_fr/1 -> fr_dugoff/4(alpha)
  [u_rl] -> rl_dugoff/2(u)
  [u_rr] -> rr_dugoff/2(u)
  lamda_fr/1 -> Gain11/1
  lamda_rl/1 -> Gain8/1
  lamda_rr/1 -> Gain9/1
  lamda_fl/1 -> Gain10/1
  alpha_rl/1 -> rl_dugoff/4(alpha)
  Gain8/1 -> rl_dugoff/3(lamda)
  Gain9/1 -> rr_dugoff/3(lamda)
  Gain10/1 -> fl_dugoff/3(lamda)
  Gain11/1 -> fr_dugoff/3(lamda)
  mu/1 -> Demux/1
  Demux/1 -> [u_fl]
  Demux/2 -> [u_fr]
  Demux/3 -> [u_rl]
  Demux/4 -> [u_rr]
  Fz_rl/1 -> rl_dugoff/1(Fz)
  Fz_fr/1 -> fr_dugoff/1(Fz)
  fl_dugoff/4(Fy) -> Fy_fl/1
  fl_dugoff/3(Fx) -> Fx_fl/1
  fr_dugoff/4(Fy) -> Fy_fr/1
  fr_dugoff/3(Fx) -> Fx_fr/1
  rl_dugoff/4(Fy) -> Fy_rl/1
  rl_dugoff/3(Fx) -> Fx_rl/1
  rr_dugoff/4(Fy) -> Fy_rr/1
  rr_dugoff/3(Fx) -> Fx_rr/1

== system tractor_mu2018/PID_Controller//直线循迹/Enabled Subsystem ==
  note: DOB:仿真步长Ts=0.001，时间常数Tao=0.1
      | 如需部署到实车需要根据实车采样频率调整
  yaw_ref : Inport
  yaw : Inport  Port=2
  beta : Inport  Port=3
  omega : Inport  Port=4
  Enable : EnablePort  StatesWhenEnabling=reset
  5500/3000 : simulink/Continuous/PID Controller  Controller=PID  Form=Parallel  TimeDomain=Discrete-time  SampleTime=-1  IntegratorMethod=Forward Euler  FilterMethod=Forward Euler  ControllerParametersSource=internal  P=5500  I=3500  D=0  N=100  UseFilter=on  TunerSelectOption=Transfer Function Based (PID Tuner App)  InitialConditionSource=internal  InitialConditionForIntegrator=0  InitialConditionForFilter=0  DifferentiatorICPrevScaledInput=0  ExternalReset=none  TrackingMode=off  Kt=1  LimitOutput=off  UpperSaturationLimit=inf  LowerSaturationLimit=-inf  LinearizeAsGain=on  AntiWindupMode=none  Kb=1  POutMin=[]  POutMax=[]  IOutMin=[]  IOutMax=[]  DOutMin=[]  DOutMax=[]  NOutMin=[]  NOutMax=[]  SumOutMin=[]  SumOutMax=[]  SaturationOutMin=[]  SaturationOutMax=[]  PParamMin=[]  PParamMax=[]  IParamMin=[]  IParamMax=[]  DParamMin=[]  DParamMax=[]  NParamMin=[]  NParamMax=[]  KbParamMin=[]  KbParamMax=[]  KtParamMin=[]  KtParamMax=[]  KbOutMin=[]  KbOutMax=[]  KtOutMin=[]  KtOutMax=[]  IntegratorOutMin=[]  IntegratorOutMax=[]  FilterOutMin=[]  FilterOutMax=[]  SumI1OutMin=[]  SumI1OutMax=[]  SumI2OutMin=[]  SumI2OutMax=[]  SumI3OutMin=[]  SumI3OutMax=[]  SumDOutMin=[]  SumDOutMax=[]  DifferentiatorOutMin=[]  DifferentiatorOutMax=[]  FilterDiffOutCoefMin=[]  FilterDiffOutCoefMax=[]  ReciprocalOutMin=[]  ReciprocalOutMax=[]  SumDenOutMin=[]  SumDenOutMax=[]  SumNumOutMin=[]  SumNumOutMax=[]  DivideOutMin=[]  DivideOutMax=[]  IntegratorContinuousStateAttributes=''  IntegratorStateMustResolveToSignalObject=off  IntegratorRTWStateStorageClass=Auto  FilterContinuousStateAttributes=''  FilterStateMustResolveToSignalObject=off  FilterRTWStateStorageClass=Auto
  Add : Sum  Inputs=+++
  Data Type Conversion : DataTypeConversion  OutDataTypeStr=single
  Data Type Conversion1 : DataTypeConversion  OutDataTypeStr=single
  Discrete Transfer Fcn : DiscreteTransferFcn  Numerator=[1-exp(-0.2)]  Denominator=[1 -exp(-0.2)]
  Gain : Gain  Gain=-1
  Gain1 : Gain  Gain=-K(1)
  Gain2 : Gain  Gain=-K(2)
  Gain3 : Gain  Gain=-K(3)
  Gain4 : Gain  Gain=3
  Gain5 : Gain  Gain=0.5
  Gain6 : Gain  Gain=180/pi
  Izr_dot : simulink/Discrete/Discrete Derivative  gainval=67536  ICPrevScaledInput=0.0  OutMin=[]  OutMax=[]  OutDataType=fixdt(1, 16)  OutScaling=2^-10  DoSatur=off
  Manual Switch : ManualSwitch
  Manual Switch1 : ManualSwitch
  Subtract : Sum  Inputs=+-
  Sum : Sum  Inputs=|+-
  Sum2 : Sum  Inputs=|+-
  Mz : Outport
  wires:
  5500/3000/1 -> Data Type Conversion1/1
  yaw_ref/1 -> Sum/1
  yaw/1 -> Sum/2
  Sum/1 -> Gain/1, Gain6/1
  Sum2/1 -> Manual Switch/2
  Discrete Transfer Fcn/1 -> Gain5/1
  Subtract/1 -> Discrete Transfer Fcn/1
  Gain3/1 -> Add/3  "eyaw"
  Gain1/1 -> Add/1  "beta"
  Izr_dot/1 -> Subtract/1
  omega/1 -> Izr_dot/1, Gain2/1
  Gain2/1 -> Add/2  "omega"
  Add/1 -> Gain4/1
  beta/1 -> Gain1/1
  Gain/1 -> Gain3/1
  Manual Switch/1 -> Manual Switch1/2
  Manual Switch1/1 -> Mz/1
  Gain4/1 -> Subtract/2, Manual Switch/1, Sum2/1
  Data Type Conversion/1 -> Sum2/2  "Mz_DOB"
  Data Type Conversion1/1 -> Manual Switch1/1  "Mz_pid"
  Gain5/1 -> Data Type Conversion/1
  Gain6/1 -> 5500/3000/1

== system tractor_mu2018/PID_Controller//直线循迹/目标航向角计算 ==
  reset : Inport
  yaw : Inport  Port=2
  omega : Inport  Port=3
  Enable : EnablePort  StatesWhenEnabling=reset
  Abs : Abs
  Add : Sum
  Constant : Constant
  Constant1 : Constant  Value=0.001
  Discrete-Time Integrator : DiscreteIntegrator  ExternalReset=rising  SampleTime=-1  ICPrevOutput=DiscIntNeverNeededParam  ICPrevScaledInput=DiscIntNeverNeededParam
  Discrete-Time Integrator1 : DiscreteIntegrator  ExternalReset=rising  SampleTime=-1  ICPrevOutput=DiscIntNeverNeededParam  ICPrevScaledInput=DiscIntNeverNeededParam
  Divide : Product  Inputs=*/
  Divide1 : Product  Inputs=*/
  Product : Product
  Saturation : Saturate  UpperLimit=999999  LowerLimit=0.1
  yaw_r : Outport
  wires:
  Constant/1 -> Divide/1
  omega/1 -> Abs/1
  Abs/1 -> Add/1
  Constant1/1 -> Add/2
  Add/1 -> Divide/2
  Divide/1 -> Discrete-Time Integrator1/1, Product/2
  yaw/1 -> Product/1
  Product/1 -> Discrete-Time Integrator/1
  Discrete-Time Integrator/1 -> Divide1/1
  Discrete-Time Integrator1/1 -> Saturation/1
  Divide1/1 -> yaw_r/1
  Saturation/1 -> Divide1/2
  reset/1 -> Discrete-Time Integrator1/2, Discrete-Time Integrator/2

== system tractor_mu2018/Subsystem/Subsystem ==
  In1 : Inport
  In2 : Inport  Port=2
  In3 : Inport  Port=3
  In4 : Inport  Port=4
  vx : Inport  Port=5
  Demux : Demux
  Gain : Gain  Gain=3.6
  MATLAB Function : MATLAB Function  TreatAsAtomicUnit=on
  Mux : Mux
  Product : Product
  Scope : Scope
  Out1 : Outport
  Out2 : Outport  Port=2
  Out3 : Outport  Port=3
  Out4 : Outport  Port=4
  wires:
  vx/1 -> Gain/1
  In1/1 -> Mux/1
  In2/1 -> Mux/2
  In3/1 -> Mux/3
  In4/1 -> Mux/4
  Demux/1 -> Out1/1
  Demux/2 -> Out2/1
  Demux/3 -> Out3/1
  Demux/4 -> Out4/1
  Gain/1 -> MATLAB Function/1(v)
  Mux/1 -> Product/1
  MATLAB Function/1(w) -> Scope/1, Product/2
  Product/1 -> Demux/1

== system tractor_mu2018/Subsystem/总纵向力估计 ==
  ax : Inport
  theta : Inport  Port=2
  T4 : Inport  Port=3
  vx : Inport  Port=4
  Abs : Abs
  Add : Sum  Inputs=++++
  Add1 : Sum  Inputs=++++
  Constant : Constant  Value=0  OutDataTypeStr=single
  Demux : Demux
  Gain : Gain  Gain=1/0.834
  Gain1 : Gain  Gain=18530*9.8
  Gain2 : Gain  Gain=0.05
  Gain3 : Gain  Gain=18530*9.8
  Gain4 : Gain  Gain=1/0.834
  Gain5 : Gain  Gain=18530
  Gain6 : Gain  Gain=1/0.94
  Gain7 : Gain  Gain=1/0.94
  Gain8 : Gain  Gain=1/3.6
  Gain9 : Gain  Gain=0
  Math Function : Math  Operator=magnitude^2  SaturateOnIntegerOverflow=on
  Min : MinMax  Inputs=2
  Sin : Trigonometry  Operator=cos
  Sin1 : Trigonometry
  Switch : Switch  Criteria=u2 > Threshold  Threshold=1
  F : Outport
  wires:
  Gain5/1 -> Add/1
  ax/1 -> Gain5/1
  theta/1 -> Sin1/1, Sin/1
  Sin/1 -> Gain1/1
  Gain1/1 -> Gain2/1
  Gain2/1 -> Add/2
  Sin1/1 -> Gain3/1
  Gain3/1 -> Add/3
  T4/1 -> Demux/1
  Demux/1 -> Gain/1
  Demux/2 -> Gain4/1
  Demux/3 -> Gain6/1
  Demux/4 -> Gain7/1
  Gain/1 -> Add1/1
  Gain4/1 -> Add1/2
  Gain6/1 -> Add1/3
  Gain7/1 -> Add1/4
  Add1/1 -> Min/2
  Add/1 -> Min/1
  Switch/1 -> F/1
  vx/1 -> Gain8/1, Abs/1
  Abs/1 -> Switch/2
  Min/1 -> Switch/1
  Constant/1 -> Switch/3
  Gain8/1 -> Math Function/1
  Math Function/1 -> Gain9/1
  Gain9/1 -> Add/4

== system tractor_mu2018/Subsystem1/Subsystem ==
  Tflref : Inport
  Tfrref : Inport  Port=2
  Trlref : Inport  Port=3
  Trrref : Inport  Port=4
  Tflbase : Inport  Port=5
  Tfrbase : Inport  Port=6
  Trlbase : Inport  Port=7
  Trrbase : Inport  Port=8
  alpha : Inport  Port=9
  Constant{,1..3} (4 alike) : Constant
  Product{,1..7} (8 alike) : Product
  Sum{,2,4,6} (4 alike) : Sum  Inputs=|+-
  Sum{1,3,5,7} (4 alike) : Sum  Inputs=|++
  alpha1 : InportShadow  Port=9
  alpha2 : InportShadow  Port=9
  alpha3 : InportShadow  Port=9
  Tfl_sh : Outport
  Tfr_sh : Outport  Port=2
  Trl_sh : Outport  Port=3
  Trr_sh : Outport  Port=4
  wires:
  Tflbase/1 -> Product/1
  Constant/1 -> Sum/1
  alpha/1 -> Sum/2, Product1/2
  Sum/1 -> Product/2
  Product/1 -> Sum1/1
  Product1/1 -> Sum1/2
  Tflref/1 -> Product1/1
  Sum1/1 -> Tfl_sh/1
  Sum3/1 -> Tfr_sh/1
  Tfrref/1 -> Product3/1
  Product3/1 -> Sum3/2
  Product2/1 -> Sum3/1
  Sum2/1 -> Product2/2
  alpha1/1 -> Product3/2, Sum2/2
  Constant1/1 -> Sum2/1
  Tfrbase/1 -> Product2/1
  Trlbase/1 -> Product4/1
  Constant2/1 -> Sum4/1
  alpha2/1 -> Sum4/2, Product5/2
  Sum4/1 -> Product4/2
  Product4/1 -> Sum5/1
  Product5/1 -> Sum5/2
  Trlref/1 -> Product5/1
  Sum5/1 -> Trl_sh/1
  Sum7/1 -> Trr_sh/1
  Trrref/1 -> Product7/1
  Product7/1 -> Sum7/2
  Product6/1 -> Sum7/1
  Sum6/1 -> Product6/2
  alpha3/1 -> Product7/2, Sum6/2
  Constant3/1 -> Sum6/1
  Trrbase/1 -> Product6/1

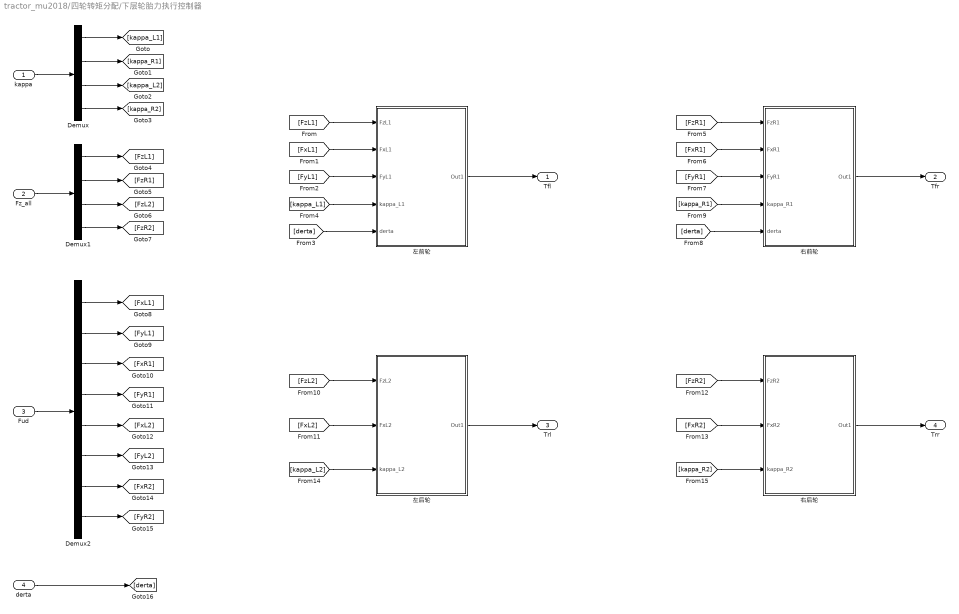
== system tractor_mu2018/四轮转矩分配/下层轮胎力执行控制器 ==
  kappa : Inport
  Fz_all : Inport  Port=2
  Fud : Inport  Port=3
  derta : Inport  Port=4
  Demux : Demux
  Demux1 : Demux
  Demux2 : Demux  Outputs=8
  右前轮 : Subsystem
  右后轮 : Subsystem
  左前轮 : Subsystem
  左后轮 : Subsystem
  Tfl : Outport
  Tfr : Outport  Port=2
  Trl : Outport  Port=3
  Trr : Outport  Port=4
  wires:
  kappa/1 -> Demux/1
  Demux/1 -> [kappa_L1]
  Demux/2 -> [kappa_R1]
  Demux/3 -> [kappa_L2]
  Demux/4 -> [kappa_R2]
  Fz_all/1 -> Demux1/1
  Demux1/1 -> [FzL1]
  Demux1/2 -> [FzR1]
  Demux1/3 -> [FzL2]
  Demux1/4 -> [FzR2]
  Fud/1 -> Demux2/1
  Demux2/1 -> [FxL1]
  Demux2/2 -> [FyL1]
  Demux2/3 -> [FxR1]
  Demux2/4 -> [FyR1]
  Demux2/6 -> [FyL2]
  Demux2/5 -> [FxL2]
  Demux2/8 -> [FyR2]
  Demux2/7 -> [FxR2]
  derta/1 -> [derta]
  左前轮/1(Out1) -> Tfl/1
  [FzL1] -> 左前轮/1(FzL1)
  [FxL1] -> 左前轮/2(FxL1)
  [FyL1] -> 左前轮/3(FyL1)
  [kappa_L1] -> 左前轮/4(kappa_L1)
  [derta] -> 左前轮/5(derta)
  [derta] -> 右前轮/5(derta)
  [kappa_R1] -> 右前轮/4(kappa_R1)
  [FyR1] -> 右前轮/3(FyR1)
  [FxR1] -> 右前轮/2(FxR1)
  [FzR1] -> 右前轮/1(FzR1)
  右前轮/1(Out1) -> Tfr/1
  [kappa_L2] -> 左后轮/3(kappa_L2)
  [FxL2] -> 左后轮/2(FxL2)
  [FzL2] -> 左后轮/1(FzL2)
  左后轮/1(Out1) -> Trl/1
  右后轮/1(Out1) -> Trr/1
  [FzR2] -> 右后轮/1(FzR2)
  [FxR2] -> 右后轮/2(FxR2)
  [kappa_R2] -> 右后轮/3(kappa_R2)

== system tractor_mu2018/总驱动力矩制定/DOB补偿 ==
  note: 仿真时间t=0.001
      | 时间常数tao=0.1
  vx : Inport
  T : Inport  Port=2
  Discrete Transfer Fcn : DiscreteTransferFcn  Numerator=[1 1]  Denominator=[201 -199]
  Discrete Derivative : simulink/Discrete/Discrete Derivative  gainval=1.0  ICPrevScaledInput=0.0  OutMin=[]  OutMax=[]  OutDataType=fixdt(1, 16)  OutScaling=2^-10  DoSatur=off
  Sum : Sum  Inputs=|-+
  m*Rf : Gain  Gain=18530*0.834
  低通LPF : DiscreteTransferFcn  Numerator=[1-0.9802]  Denominator=[1 -0.9802]
  Td_hat : Outport
  wires:
  Discrete Derivative/1 -> m*Rf/1
  vx/1 -> 低通LPF/1
  m*Rf/1 -> Sum/1
  T/1 -> Sum/2
  Sum/1 -> Discrete Transfer Fcn/1
  Discrete Transfer Fcn/1 -> Td_hat/1
  低通LPF/1 -> Discrete Derivative/1

== system tractor_mu2018/总驱动力矩制定/正常工况_高速衰减防抖 ==
  gearD : Inport
  vx : Inport  Port=2
  T0 : Inport  Port=3
  1档 : Switch  Criteria=u2 > Threshold  Threshold=14/3.6
  2档 : Switch  Criteria=u2 > Threshold  Threshold=40
  Gain14 : Gain  Gain=3.6
  Subsystem1 : Subsystem
  Switch5 : Switch  Criteria=u2 > Threshold  Threshold=1
  高速衰减冻结区 : Subsystem
  T : Outport
  wires:
  vx/1 -> 1档/2, Gain14/1
  Gain14/1 -> Subsystem1/1(v), 2档/2, 高速衰减冻结区/1(v)
  T0/1 -> 2档/3, 1档/3
  1档/1 -> Switch5/3
  Subsystem1/1(Out1) -> 2档/1
  高速衰减冻结区/1(Out1) -> 1档/1
  gearD/1 -> Switch5/2
  2档/1 -> Switch5/1
  Switch5/1 -> T/1

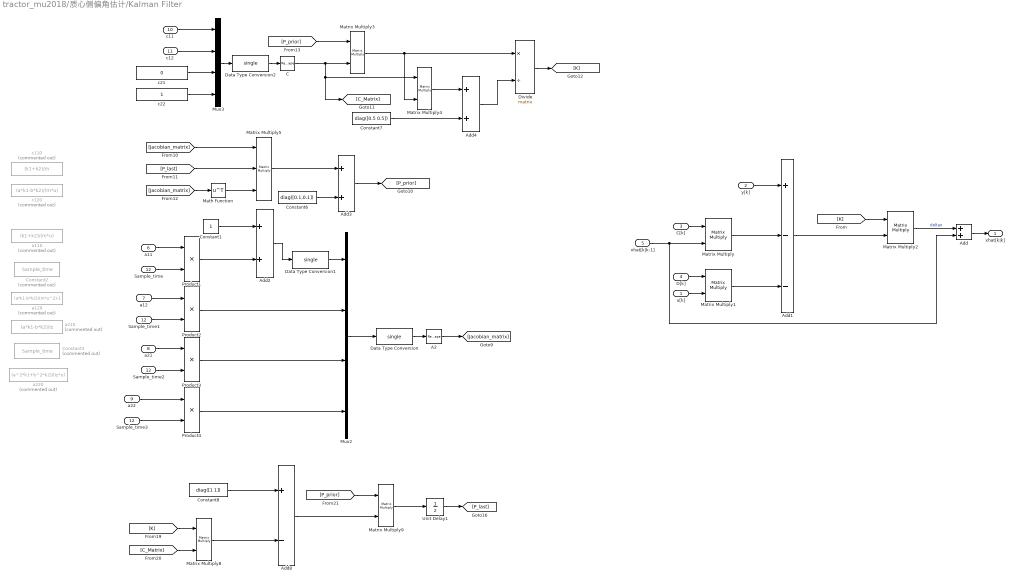
== system tractor_mu2018/质心侧偏角估计/Kalman Filter ==
  u[k] : Inport
  y[k] : Inport  Port=2
  C[k] : Inport  Port=3
  D[k] : Inport  Port=4
  xhat[k|k-1] : Inport  Port=5
  a11 : Inport  Port=6  OutDataTypeStr=single
  a12 : Inport  Port=7  OutDataTypeStr=single
  a21 : Inport  Port=8  OutDataTypeStr=single
  a22 : Inport  Port=9  OutDataTypeStr=single
  c11 : Inport  Port=10  OutDataTypeStr=single
  c12 : Inport  Port=11  OutDataTypeStr=single
  Sample_time : Inport  Port=12  OutDataTypeStr=single
  A2 : Reshape  OutputDimensionality=Customize  OutputDimensions=[2,2]
  Add{,2..4} (4 alike) : Sum
  Add1 : Sum  Inputs=+--
  Add8 : Sum  Inputs=+-
  C : Reshape  OutputDimensionality=Customize  OutputDimensions=[2,2]
  Constant1 : Constant
  Constant2 : Constant  Commented=on  Value=Sample_time
  Constant3 : Constant  Commented=on  Value=Sample_time
  Constant6 : Constant  Value=diag([0.1,0.1])
  Constant7 : Constant  Value=diag([0.5 0.5])
  Constant8 : Constant  Value=diag([1 1])
  Data Type Conversion : DataTypeConversion  OutDataTypeStr=single
  Data Type Conversion1 : DataTypeConversion  OutDataTypeStr=single
  Data Type Conversion2 : DataTypeConversion  OutDataTypeStr=single
  Divide : Product  Inputs=*/  Multiplication=Matrix(*)
  Math Function : Math  Operator=transpose  SaturateOnIntegerOverflow=on
  Matrix Multiply{,1..4,8..9} (7 alike) : Product  Multiplication=Matrix(*)
  Matrix Multiply5 : Product  Inputs=3  Multiplication=Matrix(*)
  Mux2 : Mux
  Mux3 : Mux
  Product1 : Product
  Product2 : Product
  Product3 : Product  OutDataTypeStr=single
  Product4 : Product  OutDataTypeStr=single
  Sample_time1 : InportShadow  Port=12  OutDataTypeStr=single
  Sample_time2 : InportShadow  Port=12  OutDataTypeStr=single
  Sample_time3 : InportShadow  Port=12  OutDataTypeStr=single
  Unit Delay1 : UnitDelay  SampleTime=-1  HasFrameUpgradeWarning=on
  a110 : Constant  Commented=on  Value=(k1+k2)/(m*u)
  a120 : Constant  Commented=on  Value=(a*k1-b*k2)/(m*u^2)-1
  a210 : Constant  Commented=on  Value=(a*k1-b*k2)/Iz
  a220 : Constant  Commented=on  Value=(a^2*k1+b^2*k2)/(Iz*u)
  c110 : Constant  Commented=on  Value=(k1+k2)/m
  c120 : Constant  Commented=on  Value=(a*k1-b*k2)/(m*u)
  c21 : Constant  Value=0  OutDataTypeStr=single
  c22 : Constant  OutDataTypeStr=single
  xhat[k|k] : Outport
  wires:
  Add/1 -> xhat[k|k]/1
  C[k]/1 -> Matrix Multiply/1
  xhat[k|k-1]/1 -> Matrix Multiply/2, Add/2
  D[k]/1 -> Matrix Multiply1/1
  u[k]/1 -> Matrix Multiply1/2
  y[k]/1 -> Add1/1
  Matrix Multiply/1 -> Add1/2
  Matrix Multiply1/1 -> Add1/3
  Add1/1 -> Matrix Multiply2/2
  Matrix Multiply2/1 -> Add/1  "deltax"
  Add4/1 -> Divide/2
  Matrix Multiply3/1 -> Divide/1, Matrix Multiply4/2
  c21/1 -> Mux3/3
  Matrix Multiply4/1 -> Add4/1
  c22/1 -> Mux3/4
  Mux3/1 -> Data Type Conversion2/1
  Constant7/1 -> Add4/2
  c11/1 -> Mux3/1
  [P_prior] -> Matrix Multiply3/1
  C/1 -> Matrix Multiply4/1, [C_Matrix], Matrix Multiply3/2
  Divide/1 -> [K]
  [P_last] -> Matrix Multiply5/2
  Matrix Multiply5/1 -> Add3/1
  [Jacobian_matrix] -> Math Function/1
  Math Function/1 -> Matrix Multiply5/3
  Add3/1 -> [P_prior]
  [Jacobian_matrix] -> Matrix Multiply5/1
  Constant6/1 -> Add3/2
  Sample_time2/1 -> Product3/2
  Sample_time3/1 -> Product4/2
  a12/1 -> Product2/1
  A2/1 -> [Jacobian_matrix]
  Add2/1 -> Data Type Conversion1/1
  Product1/1 -> Add2/2
  Sample_time1/1 -> Product2/2
  a22/1 -> Product4/1
  Mux2/1 -> Data Type Conversion/1
  a21/1 -> Product3/1
  Constant1/1 -> Add2/1
  [K] -> Matrix Multiply2/1
  Matrix Multiply8/1 -> Add8/2
  Constant8/1 -> Add8/1
  Unit Delay1/1 -> [P_last]
  [P_prior] -> Matrix Multiply9/1
  Add8/1 -> Matrix Multiply9/2
  Matrix Multiply9/1 -> Unit Delay1/1
  [K] -> Matrix Multiply8/1
  [C_Matrix] -> Matrix Multiply8/2
  a11/1 -> Product1/1
  c12/1 -> Mux3/2
  Sample_time/1 -> Product1/2
  Product2/1 -> Mux2/2
  Product3/1 -> Mux2/3
  Product4/1 -> Mux2/4
  Data Type Conversion/1 -> A2/1
  Data Type Conversion1/1 -> Mux2/1
  Data Type Conversion2/1 -> C/1

== system tractor_mu2018/质心侧偏角估计/Observer ==
  note: A*xhat+B*u+L*(yMeas-yHat)
      | or
      | A*xhat+B*u
  u[k] : Inport
  y[k] : Inport  Port=2
  A[k] : Inport  Port=3
  B[k] : Inport  Port=4
  C[k] : Inport  Port=5
  D[k] : Inport  Port=6
  L[k] : Inport  Port=7
  xhat[k|k-1] : Inport  Port=8
  Add : Sum  Inputs=+++
  Matrix Multiply : Product  Multiplication=Matrix(*)
  Matrix Multiply1 : Product  Multiplication=Matrix(*)
  Reshape : Reshape
  Subsystem : Subsystem
  x[k+1|k] : Outport
  wires:
  B[k]/1 -> Matrix Multiply/1
  u[k]/1 -> Subsystem/6(u[k]), Matrix Multiply/2
  A[k]/1 -> Matrix Multiply1/1
  xhat[k|k-1]/1 -> Matrix Multiply1/2, Subsystem/4(xhat[k|k-1])
  L[k]/1 -> Subsystem/1(L[k])
  y[k]/1 -> Subsystem/2(y[k])
  C[k]/1 -> Subsystem/3(C[k])
  D[k]/1 -> Subsystem/5(D[k])
  Matrix Multiply/1 -> Add/1
  Matrix Multiply1/1 -> Add/2
  Subsystem/1(L*(y[k]-yhat[k|k-1])) -> Add/3
  Add/1 -> Reshape/1
  Reshape/1 -> x[k+1|k]/1

== system tractor_mu2018/质心侧偏角滑模观测器估计/Subsystem ==
  Avz_Carsim : Inport
  vx : Inport  Port=2
  delta_f : Inport  Port=3
  Atan : Trigonometry  Operator=atan
  Constant : Constant  Value=0.1
  Divide : Product  Inputs=*/
  Gain1 : Gain  Gain=L1
  Gain2 : Gain  Gain=L2
  MATLAB Function : MATLAB Function  TreatAsAtomicUnit=on  SystemSampleTime=0.005
  Scope1 : Scope
  Scope2 : Scope
  Subsystem : Subsystem
  Sum : Sum  Inputs=|+-
  Sum1 : Sum  Inputs=|++
  Sum2 : Sum  Inputs=|++
  Switch : Switch  Criteria=u2 > Threshold  Threshold=0.1
  gamma_hat : DiscreteIntegrator  SampleTime=-1  ICPrevOutput=DiscIntNeverNeededParam  ICPrevScaledInput=DiscIntNeverNeededParam
  vy_hat : DiscreteIntegrator  SampleTime=-1  ICPrevOutput=DiscIntNeverNeededParam  ICPrevScaledInput=DiscIntNeverNeededParam
  beta_est : Outport
  gamma_est : Outport  Port=2
  vy_hat_output : Outport  Port=3
  wires:
  Avz_Carsim/1 -> Sum/1
  Sum/1 -> Subsystem/1(error)
  MATLAB Function/1(d_vy_model) -> Sum1/2
  gamma_hat/1 -> Scope1/1, MATLAB Function/4(gamma_hat), gamma_est/1, Sum/2
  vx/1 -> Scope2/1, Switch/1, Switch/2
  Constant/1 -> Switch/3
  vy_hat/1 -> vy_hat_output/1, Divide/1, MATLAB Function/3(vy_hat)
  Switch/1 -> Divide/2, MATLAB Function/1(vx)
  Subsystem/1(v_STA) -> Gain2/1, Gain1/1
  delta_f/1 -> MATLAB Function/2(delta_f)
  Divide/1 -> Atan/1
  Gain1/1 -> Sum1/1
  Gain2/1 -> Sum2/1
  MATLAB Function/2(d_gamma_model) -> Sum2/2
  Atan/1 -> beta_est/1
  Sum1/1 -> vy_hat/1
  Sum2/1 -> gamma_hat/1

== system tractor_mu2018/质心侧偏角滑模观测器估计/Subsystem1 ==
  Avz_Carsim : Inport
  vx : Inport  Port=2
  delta_f : Inport  Port=3
  Atan : Trigonometry  Operator=atan
  Constant : Constant  Value=0.1
  Divide : Product  Inputs=*/
  Gain : Gain  Gain=1/Phi
  Gain1 : Gain  Gain=L1
  Gain2 : Gain  Gain=L2
  MATLAB Function : MATLAB Function  TreatAsAtomicUnit=on  SystemSampleTime=0.005
  Saturation : Saturate  UpperLimit=1  LowerLimit=-1
  Scope1 : Scope
  Scope2 : Scope
  Sum : Sum  Inputs=|+-
  Sum1 : Sum  Inputs=|++
  Sum2 : Sum  Inputs=|++
  Switch : Switch  Criteria=u2 > Threshold  Threshold=0.1
  gamma_hat : Integrator
  vy_hat : Integrator
  beta_est : Outport
  gamma_est : Outport  Port=2
  vy_hat_output : Outport  Port=3
  wires:
  Gain/1 -> Saturation/1
  Avz_Carsim/1 -> Sum/1
  Sum/1 -> Gain/1
  MATLAB Function/1(d_vy_model) -> Sum1/2
  gamma_hat/1 -> Scope1/1, MATLAB Function/4(gamma_hat), gamma_est/1, Sum/2
  vx/1 -> Scope2/1, Switch/1, Switch/2
  Constant/1 -> Switch/3
  vy_hat/1 -> vy_hat_output/1, Divide/1, MATLAB Function/3(vy_hat)
  Switch/1 -> Divide/2, MATLAB Function/1(vx)
  Saturation/1 -> Gain2/1, Gain1/1
  delta_f/1 -> MATLAB Function/2(delta_f)
  Divide/1 -> Atan/1
  Gain1/1 -> Sum1/1
  Gain2/1 -> Sum2/1
  MATLAB Function/2(d_gamma_model) -> Sum2/2
  Atan/1 -> beta_est/1
  Sum1/1 -> vy_hat/1
  Sum2/1 -> gamma_hat/1

== system tractor_mu2018/驱动防滑模块/Subsystem ==
  lamda1 : Inport
  p : Inport  Port=2
  i : Inport  Port=3
  b : Inport  Port=4
  Constant : Constant  Value=0.2
  PID Controller : simulink/Continuous/PID Controller  Controller=PI  Form=Parallel  TimeDomain=Discrete-time  SampleTime=-1  IntegratorMethod=Forward Euler  FilterMethod=Forward Euler  ControllerParametersSource=external  P=5000  I=3000  D=0  N=100  UseFilter=on  TunerSelectOption=Transfer Function Based (PID Tuner App)  InitialConditionSource=internal  InitialConditionForIntegrator=0  InitialConditionForFilter=0  DifferentiatorICPrevScaledInput=0  ExternalReset=none  TrackingMode=off  Kt=1  LimitOutput=on  UpperSaturationLimit=0  LowerSaturationLimit=-30000  LinearizeAsGain=on  AntiWindupMode=clamping  Kb=1  POutMin=[]  POutMax=[]  IOutMin=[]  IOutMax=[]  DOutMin=[]  DOutMax=[]  NOutMin=[]  NOutMax=[]  SumOutMin=[]  SumOutMax=[]  SaturationOutMin=[]  SaturationOutMax=[]  PParamMin=[]  PParamMax=[]  IParamMin=[]  IParamMax=[]  DParamMin=[]  DParamMax=[]  NParamMin=[]  NParamMax=[]  KbParamMin=[]  KbParamMax=[]  KtParamMin=[]  KtParamMax=[]  KbOutMin=[]  KbOutMax=[]  KtOutMin=[]  KtOutMax=[]  IntegratorOutMin=[]  IntegratorOutMax=[]  FilterOutMin=[]  FilterOutMax=[]  SumI1OutMin=[]  SumI1OutMax=[]  SumI2OutMin=[]  SumI2OutMax=[]  SumI3OutMin=[]  SumI3OutMax=[]  SumDOutMin=[]  SumDOutMax=[]  DifferentiatorOutMin=[]  DifferentiatorOutMax=[]  FilterDiffOutCoefMin=[]  FilterDiffOutCoefMax=[]  ReciprocalOutMin=[]  ReciprocalOutMax=[]  SumDenOutMin=[]  SumDenOutMax=[]  SumNumOutMin=[]  SumNumOutMax=[]  DivideOutMin=[]  DivideOutMax=[]  IntegratorContinuousStateAttributes=''  IntegratorStateMustResolveToSignalObject=off  IntegratorRTWStateStorageClass=Auto  FilterContinuousStateAttributes=''  FilterStateMustResolveToSignalObject=off  FilterRTWStateStorageClass=Auto
  Saturation : Saturate  UpperLimit=30000  LowerLimit=-30000
  Sum4 : Sum  Inputs=|+-
  dT1 : Outport
  wires:
  Sum4/1 -> PID Controller/1
  lamda1/1 -> Sum4/2
  PID Controller/1 -> Saturation/1  "dT1"
  p/1 -> PID Controller/2
  i/1 -> PID Controller/3
  Constant/1 -> Sum4/1
  Saturation/1 -> dT1/1
